simulink model "XAERO03_reference"  (R2025a)
settings: Solver=FixedStepDiscrete  StartTime=0  StopTime=30  FixedStep=0.01  RelTol=1e-3
undefined symbols (not defined in the file): airspeed_reference, altitude_reference, command_time, gust_heading, gust_speed, gust_time, heading_change, initial_airspeed_offset, initial_altitude_offset
Description:
  | Independent causal reference with NED rigid-body motion, relative-wind aerodynamics, bounded finite-rate actuators, measured-state feedback and same-path force/moment logs.
settings Model: Creator=SimuVerity Contributors  LastModifiedBy=SimuVerity Contributors
settings DataIOCC: SignalLogging=off

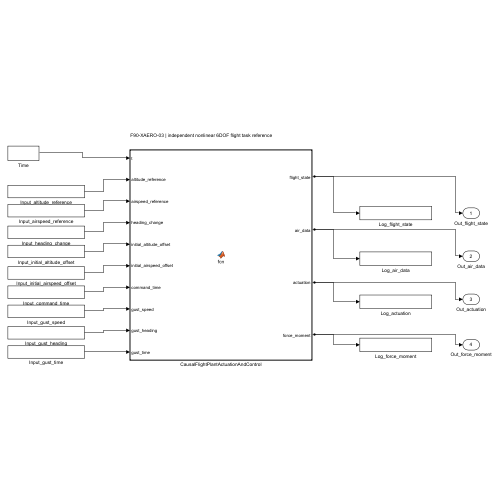
[thumbnail: Simulink's stored preview of the top-level diagram]
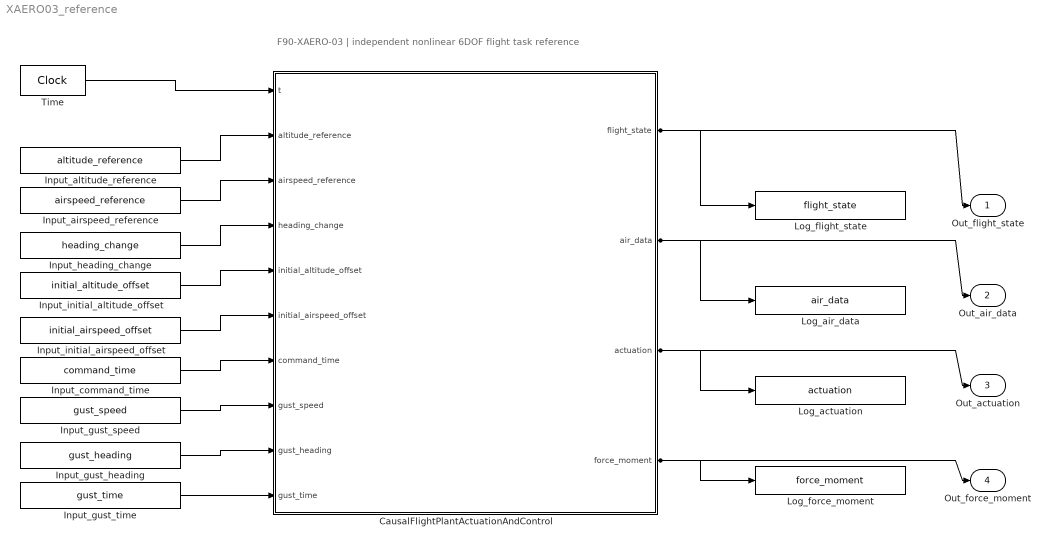
== system XAERO03_reference ==
  note: F90-XAERO-03 | independent nonlinear 6DOF flight task reference
  CausalFlightPlantActuationAndControl : MATLAB Function  TreatAsAtomicUnit=on
  Input_airspeed_reference : Constant  Value=airspeed_reference
  Input_altitude_reference : Constant  Value=altitude_reference
  Input_command_time : Constant  Value=command_time
  Input_gust_heading : Constant  Value=gust_heading
  Input_gust_speed : Constant  Value=gust_speed
  Input_gust_time : Constant  Value=gust_time
  Input_heading_change : Constant  Value=heading_change
  Input_initial_airspeed_offset : Constant  Value=initial_airspeed_offset
  Input_initial_altitude_offset : Constant  Value=initial_altitude_offset
  Log_actuation : ToWorkspace  VariableName=actuation  SaveFormat=Timeseries  SampleTime=-1
  Log_air_data : ToWorkspace  VariableName=air_data  SaveFormat=Timeseries  SampleTime=-1
  Log_flight_state : ToWorkspace  VariableName=flight_state  SaveFormat=Timeseries  SampleTime=-1
  Log_force_moment : ToWorkspace  VariableName=force_moment  SaveFormat=Timeseries  SampleTime=-1
  Time : DigitalClock  SampleTime=0.01
  Out_flight_state : Outport
  Out_air_data : Outport  Port=2
  Out_actuation : Outport  Port=3
  Out_force_moment : Outport  Port=4
  wires:
  Time/1 -> CausalFlightPlantActuationAndControl/1(t)
  Input_altitude_reference/1 -> CausalFlightPlantActuationAndControl/2(altitude_reference)
  Input_airspeed_reference/1 -> CausalFlightPlantActuationAndControl/3(airspeed_reference)
  Input_heading_change/1 -> CausalFlightPlantActuationAndControl/4(heading_change)
  Input_initial_altitude_offset/1 -> CausalFlightPlantActuationAndControl/5(initial_altitude_offset)
  Input_initial_airspeed_offset/1 -> CausalFlightPlantActuationAndControl/6(initial_airspeed_offset)
  Input_command_time/1 -> CausalFlightPlantActuationAndControl/7(command_time)
  Input_gust_speed/1 -> CausalFlightPlantActuationAndControl/8(gust_speed)
  Input_gust_heading/1 -> CausalFlightPlantActuationAndControl/9(gust_heading)
  Input_gust_time/1 -> CausalFlightPlantActuationAndControl/10(gust_time)
  CausalFlightPlantActuationAndControl/1(flight_state) -> Log_flight_state/1, Out_flight_state/1
  CausalFlightPlantActuationAndControl/2(air_data) -> Log_air_data/1, Out_air_data/1
  CausalFlightPlantActuationAndControl/3(actuation) -> Log_actuation/1, Out_actuation/1
  CausalFlightPlantActuationAndControl/4(force_moment) -> Log_force_moment/1, Out_force_moment/1

== matlab function XAERO03_reference/CausalFlightPlantActuationAndControl ==
  data: t input; flight_state output; altitude_reference input; airspeed_reference input; heading_change input; initial_altitude_offset input; initial_airspeed_offset input; command_time input; gust_speed input; gust_heading input; gust_time input; air_data output; actuation output; force_moment output
function [flight_state,air_data,actuation,force_moment] = fcn( ...
    t,altitude_reference,airspeed_reference,heading_change, ...
    initial_altitude_offset,initial_airspeed_offset,command_time, ...
    gust_speed,gust_heading,gust_time)
%#codegen
persistent position bodyVelocity euler omega actuator

dt = 0.01;
mass = 9295.438666;
area = 27.870912;
span = 9.144;
chord = 3.450336;
gravity = 9.806;
inertia = [ ...
    12874.844646 0 1331.412957; ...
    0 75673.607738 0; ...
    1331.412957 0 85552.095321];
lower = [4448.22;-.436332313;-.375245789;-.523598776;0];
upper = [84516.18;.436332313;.375245789;.523598776;.436332313];
rate = [44482.2;1.047197551;1.396263402;2.094395102;.436332313];

if isempty(position) || t < .5*dt
    altitude0 = altitude_reference+initial_altitude_offset;
    speed0 = airspeed_reference+initial_airspeed_offset;
    [alpha0,elevator0,lef0,thrust0] = trim_values( ...
        altitude0,speed0,mass,area,gravity,lower,upper);
    position = [0;0;-altitude0];
    bodyVelocity = [speed0*cos(alpha0);0;speed0*sin(alpha0)];
    euler = [0;alpha0;0];
    omega = zeros(3,1);
    actuator = [thrust0;elevator0;0;0;lef0];
end

phi = euler(1);
theta = euler(2);
psi = euler(3);
dcm = body_to_ned(phi,theta,psi);
inertialVelocity = dcm*bodyVelocity;
altitude = -position(3);

gustNed = zeros(3,1);
if t >= gust_time && t < gust_time+1.5
    heading = gust_heading*pi/180;
    gustNed(1) = gust_speed*cos(heading);
    gustNed(2) = gust_speed*sin(heading);
end
relativeBodyVelocity = dcm'*(inertialVelocity-gustNed);
trueAirspeed = max(norm(relativeBodyVelocity),30);
alpha = atan2(relativeBodyVelocity(3),relativeBodyVelocity(1));
beta = asin(clip(relativeBodyVelocity(2)/trueAirspeed,-.99,.99));
[density,soundSpeed] = atmosphere(altitude);
dynamicPressure = .5*density*trueAirspeed^2;

if t >= command_time, headingReference = heading_change;
else, headingReference = 0;
end
headingError = wrap_angle(headingReference-psi);
rollReference = clip(1.15*headingError,-.50,.50);
altitudeError = altitude_reference-altitude;
downVelocity = inertialVelocity(3);
[alphaReference,~,~,~] = trim_values( ...
    altitude,airspeed_reference,mass,area,gravity,lower,upper);
pitchReference = clip( ...
    alphaReference+0.0010580000000000001*altitudeError+0.022800000000000001*downVelocity,-.30,.38);
[~,elevatorTrim,~,~] = trim_values( ...
    altitude,trueAirspeed,mass,area,gravity,lower,upper);

estimatedLift = .15+4.5*alpha-.7*actuator(2)+.35*actuator(5);
estimatedDrag = .025+.18*estimatedLift^2+.06*beta^2+ ...
    .02*(actuator(2)/upper(2))^2+ ...
    .01*(actuator(3)/upper(3))^2;
trimThrust = dynamicPressure*area*estimatedDrag;
command = zeros(5,1);
command(1) = trimThrust+2208*(airspeed_reference-trueAirspeed);
command(2) = elevatorTrim-1.4724999999999999*(pitchReference-theta)+0.74099999999999999*omega(2);
command(3) = 2.4*(rollReference-phi)-.55*omega(1);
command(4) = 1.8*beta+.35*omega(3)-.12*headingError;
command(5) = 2*max(alpha,0);
command = clip(command,lower,upper);

thrust = actuator(1);
elevator = actuator(2);
aileron = actuator(3);
rudder = actuator(4);
lef = actuator(5);
pHat = omega(1)*span/(2*trueAirspeed);
qHat = omega(2)*chord/(2*trueAirspeed);
rHat = omega(3)*span/(2*trueAirspeed);
liftCoefficient = .15+4.5*alpha-.7*elevator+.35*lef+1.8*qHat;
dragCoefficient = .025+.18*liftCoefficient^2+.06*beta^2+ ...
    .02*(elevator/upper(2))^2+.01*(aileron/upper(3))^2;
sideCoefficient = -.9*beta-.35*rHat+.20*rudder+.08*aileron;
lift = dynamicPressure*area*liftCoefficient;
drag = dynamicPressure*area*dragCoefficient;
aerodynamicForce = [ ...
    -drag*cos(alpha)+lift*sin(alpha); ...
    dynamicPressure*area*sideCoefficient; ...
    -drag*sin(alpha)-lift*cos(alpha)];

rollCoefficient = -.12*beta-.48*pHat+.12*aileron+.04*rudder;
pitchCoefficient = ...
    .04-.9*alpha-1.1*qHat-1.3*elevator+.12*lef;
yawCoefficient = ...
    .18*beta-.38*rHat-.10*rudder+.025*aileron;
aerodynamicMoment = [ ...
    dynamicPressure*area*span*rollCoefficient; ...
    dynamicPressure*area*chord*pitchCoefficient; ...
    dynamicPressure*area*span*yawCoefficient];

gravityBody = dcm'*[0;0;mass*gravity];
totalForce = aerodynamicForce+[thrust;0;0]+gravityBody;
totalMoment = aerodynamicMoment;
bodyAcceleration = totalForce/mass-cross(omega,bodyVelocity);
angularAcceleration = inertia \ ( ...
    totalMoment-cross(omega,inertia*omega));

cosineTheta = sign(cos(theta))*max(abs(cos(theta)),.15);
if cosineTheta == 0, cosineTheta = .15; end
eulerMatrix = [ ...
    1 sin(phi)*tan(theta) cos(phi)*tan(theta); ...
    0 cos(phi) -sin(phi); ...
    0 sin(phi)/cosineTheta cos(phi)/cosineTheta];
eulerDerivative = eulerMatrix*omega;

flight_state = [ ...
    position(1) position(2) altitude inertialVelocity' ...
    trueAirspeed alpha beta euler' omega'];
air_data = [ ...
    density dynamicPressure trueAirspeed/soundSpeed gustNed'];
actuation = [command' actuator'];
force_moment = [ ...
    aerodynamicForce' aerodynamicMoment' ...
    totalForce' totalMoment'];

position = position+dt*inertialVelocity;
bodyVelocity = bodyVelocity+dt*bodyAcceleration;
euler = euler+dt*eulerDerivative;
euler(3) = wrap_angle(euler(3));
omega = omega+dt*angularAcceleration;
actuator = clip( ...
    actuator+clip(command-actuator,-rate*dt,rate*dt),lower,upper);
end

function dcm = body_to_ned(phi,theta,psi)
cphi = cos(phi); sphi = sin(phi);
ctheta = cos(theta); stheta = sin(theta);
cpsi = cos(psi); spsi = sin(psi);
dcm = [ ...
    ctheta*cpsi, ...
    sphi*stheta*cpsi-cphi*spsi, ...
    cphi*stheta*cpsi+sphi*spsi; ...
    ctheta*spsi, ...
    sphi*stheta*spsi+cphi*cpsi, ...
    cphi*stheta*spsi-sphi*cpsi; ...
    -stheta,sphi*ctheta,cphi*ctheta];
end

function [density,soundSpeed] = atmosphere(altitude)
h = max(altitude,0);
density = 1.225*exp(-h/8500);
temperature = max(216.65,288.15-.0065*h);
soundSpeed = sqrt(1.4*287.05*temperature);
end

function [alpha,elevator,lef,thrust] = trim_values( ...
        altitude,speed,mass,area,gravity,lower,upper)
[density,~] = atmosphere(altitude);
dynamicPressure = .5*density*speed^2;
alpha = .08;
for index = 1:20 %#ok<NASGU>
    lef = clip(2*alpha,0,upper(5));
    elevator = (.04-.9*alpha+.12*lef)/1.3;
    liftCoefficient = .15+4.5*alpha-.7*elevator+.35*lef;
    alpha = alpha+(mass*gravity/(dynamicPressure*area)- ...
        liftCoefficient)/5;
end
alpha = clip(alpha,-.10,.35);
lef = clip(2*alpha,0,upper(5));
elevator = clip( ...
    (.04-.9*alpha+.12*lef)/1.3,lower(2),upper(2));
liftCoefficient = .15+4.5*alpha-.7*elevator+.35*lef;
dragCoefficient = ...
    .025+.18*liftCoefficient^2+.02*(elevator/upper(2))^2;
thrust = clip( ...
    dynamicPressure*area*dragCoefficient,lower(1),upper(1));
end

function value = wrap_angle(value)
value = mod(value+pi,2*pi)-pi;
end

function value = clip(value,lower,upper)
value = min(max(value,lower),upper);
end
